simulink model "fir_col_test"  (Simulink 7.2)
settings: Solver=VariableStepDiscrete  StartTime=0.0  StopTime=100  RelTol=1e-3
libraries: xbsIndex_r4 x23, casper_library_downconverter x4
settings Model: Creator=User  LastModifiedBy=root
settings OptimizationCC: InitFltsAndDblsToZero=on
settings DebuggingCC: SaveWithDisabledLinksMsg=none  SaveWithParameterizedLinksMsg=none

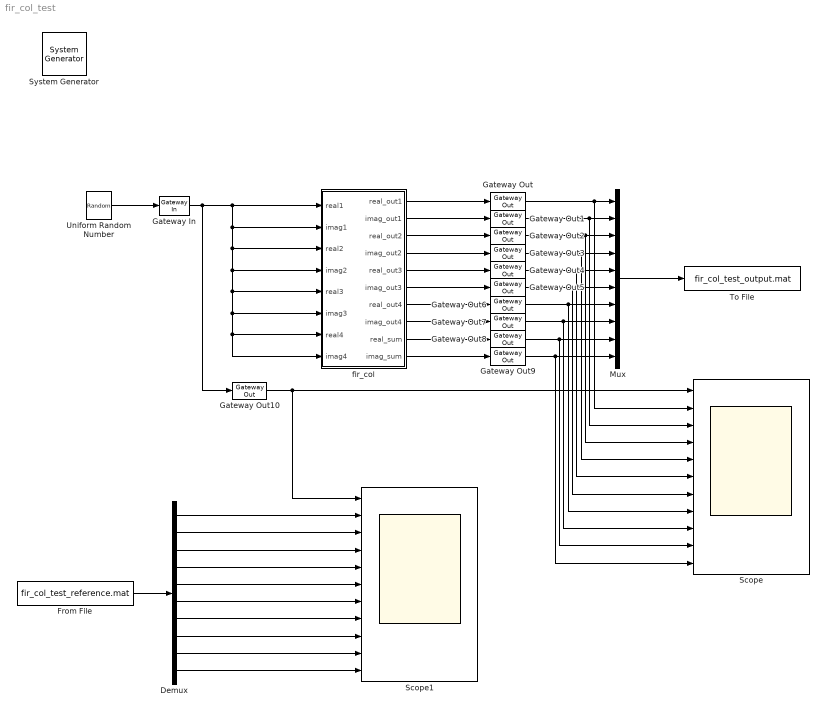
== system fir_col_test ==
  " System Generator" : xbsIndex_r4/ System Generator  Tag=genX  SystemSampleTime=-1  xilinxfamily=Virtex4  part=xc4vsx35  speed=-10  package=ff668  synthesis_tool=XST  clock_wrapper=Clock Enables  directory=./netlist  testbench=off  simulink_period=1  sysclk_period=100  dcm_input_clock_period=100  incr_netlist=off  trim_vbits=Everywhere in SubSystem  dbl_ovrd=According to Block Masks  core_generation=According to Block Masks  run_coregen=off  deprecated_control=off  eval_field=0  block_type=sysgen
      settings: block_version=10.1.1
  Demux : Demux  Outputs=10
  From File : FromFile  FileName=fir_col_test_reference.mat  SampleTime=1
  Gateway In : xbsIndex_r4/Gateway In  arith_type="Signed  (2's comp)"  n_bits=16  bin_pt=15  quantization="Round  (unbiased: +/- Inf)"  overflow=Saturate  period=1  dbl_ovrd=off  timing_constraint=None  locs_specified=off  LOCs={}  hdl_port=on  block_type=gatewayin
      settings: infoedit="Gateway in block.  Converts inputs of type Simulink integer, double and fixed point to  Xilinx fixed point type.<P><P>Hardware notes:  In hardware these blocks become top level input ports."  block_version=10.1.1
  Gateway Out{,1..10} (11 alike) : xbsIndex_r4/Gateway Out  hdl_port=on  timing_constraint=None  locs_specified=off  LOCs={}  block_type=gatewayout
      settings: infoedit="Gateway out block.  Converts Xilinx fixed point inputs into ouputs of type Simulink integer, double, or fixed point.<P><P>Hardware notes:  In hardware these blocks become top level output ports or are discarded, depending on how they are configured."  block_version=10.1.1
  Mux : Mux  Inputs=10
  Scope : Scope  NumInputPorts=11
      settings: YMin=-1~-1~-1~-1~-1~-1~-1~-1~-1~-5~-5  YMax=1~1~1~1~1~1~1~1~1~5~5
  Scope1 : Scope  NumInputPorts=11
      settings: YMin=-1~-1~-1~-1~-1~-1~-1~-1~-1~-5~-5  YMax=1~1~1~1~1~1~1~1~1~5~5
  To File : ToFile  Filename=fir_col_test_output.mat  MatrixName=output
  Uniform Random Number : UniformRandomNumber  SampleTime=0
  fir_col : Subsystem  AncestorBlock=casper_library_downconverter/fir_col  mask(fir_col){n_inputs=4, coeff=getfield( getfield( get_param( gcb,'UserData' ), 'parameters'),'coeff'), add_latency=4, mult_latency=3, coeff_bit_width=18, coeff_bin_pt=17, first_stage_hdl=on, adder_imp=Fabric}
      mask prompts: n_inputs "Inputs"; coeff "Coefficients"; add_latency "Add latency"; mult_latency "Mult Latency"; coeff_bit_width "Coefficient bit width"; coeff_bin_pt "Coefficient binary point"; first_stage_hdl "Implement first stage of adder trees on output as behavioural HDL"; adder_imp "Adder implementation"
      mask init:
      | fir_col_init(gcb, ...
      |     'n_inputs', n_inputs,...
      |     'coeff', coeff, ...
      |     'mult_latency', mult_latency, ...
      |     'add_latency', add_latency, ...
      |     'coeff_bit_width', coeff_bit_width, ...
      |     'coeff_bin_pt', coeff_bin_pt, ...
      |     'first_stage_hdl', first_stage_hdl, ...
      |     'adder_imp', adder_imp);
      mask Help: eval('xlWeb(''http://casper.berkeley.edu/wiki/Fir_col'')')
      mask StyleString: edit,edit,edit,edit,edit,edit,checkbox,popup(Behavioral|Fabric|DSP48)
  wires:
  Uniform Random Number/1 -> Gateway In/1
  Gateway In/1 -> fir_col/8(imag4), fir_col/7(real4), fir_col/6(imag3), fir_col/5(real3), fir_col/4(imag2), fir_col/3(real2), fir_col/2(imag1), fir_col/1(real1), Gateway Out10/1
  fir_col/1(real_out1) -> Gateway Out/1
  fir_col/2(imag_out1) -> Gateway Out1/1
  fir_col/3(real_out2) -> Gateway Out2/1
  fir_col/4(imag_out2) -> Gateway Out3/1
  fir_col/5(real_out3) -> Gateway Out4/1
  fir_col/6(imag_out3) -> Gateway Out5/1
  fir_col/7(real_out4) -> Gateway Out6/1
  fir_col/8(imag_out4) -> Gateway Out7/1
  fir_col/9(real_sum) -> Gateway Out8/1
  fir_col/10(imag_sum) -> Gateway Out9/1
  Gateway Out/1 -> Mux/1, Scope/2
  Gateway Out1/1 -> Mux/2, Scope/3
  Gateway Out2/1 -> Mux/3, Scope/4
  Gateway Out3/1 -> Mux/4, Scope/5
  Gateway Out4/1 -> Mux/5, Scope/6
  Gateway Out5/1 -> Mux/6, Scope/7
  Gateway Out6/1 -> Mux/7, Scope/8
  Gateway Out7/1 -> Mux/8, Scope/9
  Gateway Out8/1 -> Mux/9, Scope/10
  Gateway Out9/1 -> Mux/10, Scope/11
  Mux/1 -> To File/1
  Gateway Out10/1 -> Scope/1, Scope1/1
  From File/1 -> Demux/1
  Demux/1 -> Scope1/2
  Demux/2 -> Scope1/3
  Demux/3 -> Scope1/4
  Demux/4 -> Scope1/5
  Demux/5 -> Scope1/6
  Demux/6 -> Scope1/7
  Demux/7 -> Scope1/8
  Demux/8 -> Scope1/9
  Demux/9 -> Scope1/10
  Demux/10 -> Scope1/11

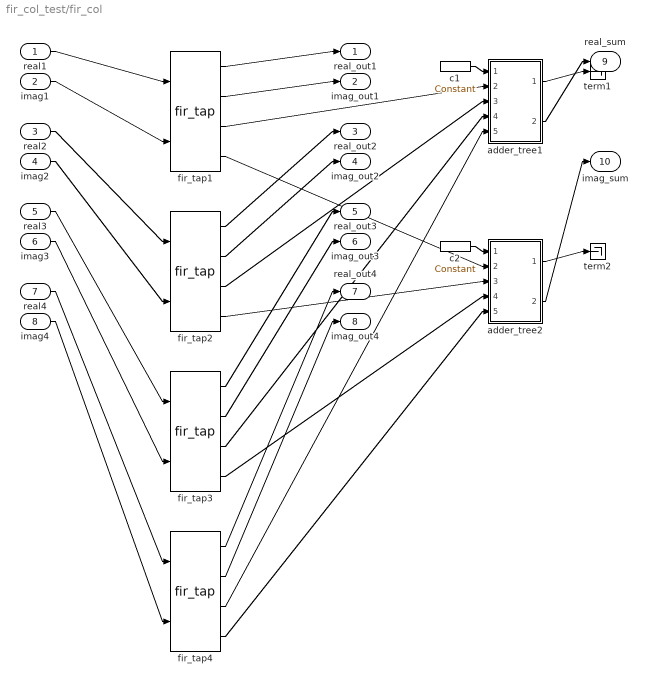
== system fir_col_test/fir_col ==
  real1 : Inport
  imag1 : Inport  Port=2
  real2 : Inport  Port=3
  imag2 : Inport  Port=4
  real3 : Inport  Port=5
  imag3 : Inport  Port=6
  real4 : Inport  Port=7
  imag4 : Inport  Port=8
  adder_tree1 : Subsystem  AncestorBlock=casper_library_misc/adder_tree  mask(adder_tree){n_inputs=4, latency=4, adder_imp=Fabric, first_stage_hdl=on}
      mask prompts: n_inputs "Number of Inputs"; latency "Add Latency"; adder_imp "Adder implementation"; first_stage_hdl "Use behavioural HDL for first stage of adders"
      mask help:
      | Sums all inputs using a tree of adds and delays.
      |
      | Number of inputs: The number of inputs to the block to be summed
      | Add latency: The number of clock cycles to perform one addition (affects timing)..
      | Adder implementation: choice of fabric or DSP48E core, or behavioral HDL
      | Use behavioural HDL for first stage of adders: Causes the first stage of adders to be absorbed into DSP blocks if multipliers precede them (Virtex 5). Overrides Adder implementation
      mask init:
      | adder_tree_init(gcb, ...
      |     'n_inputs', n_inputs, ...
      |     'latency', latency, ...
      |     'adder_imp', adder_imp, ...
      |     'first_stage_hdl', first_stage_hdl);
      settings: AttributesFormatString=latency 8
      mask Help: eval('xlWeb(''http://casper.berkeley.edu/wiki/Adder_tree'')')
      mask StyleString: edit,edit,popup(Behavioral|Fabric|DSP48),checkbox
  adder_tree2 : Subsystem  AncestorBlock=casper_library_misc/adder_tree  mask(adder_tree){n_inputs=4, latency=4, adder_imp=Fabric, first_stage_hdl=on}
      mask prompts: n_inputs "Number of Inputs"; latency "Add Latency"; adder_imp "Adder implementation"; first_stage_hdl "Use behavioural HDL for first stage of adders"
      mask help:
      | Sums all inputs using a tree of adds and delays.
      |
      | Number of inputs: The number of inputs to the block to be summed
      | Add latency: The number of clock cycles to perform one addition (affects timing)..
      | Adder implementation: choice of fabric or DSP48E core, or behavioral HDL
      | Use behavioural HDL for first stage of adders: Causes the first stage of adders to be absorbed into DSP blocks if multipliers precede them (Virtex 5). Overrides Adder implementation
      mask init:
      | adder_tree_init(gcb, ...
      |     'n_inputs', n_inputs, ...
      |     'latency', latency, ...
      |     'adder_imp', adder_imp, ...
      |     'first_stage_hdl', first_stage_hdl);
      settings: AttributesFormatString=latency 8
      mask Help: eval('xlWeb(''http://casper.berkeley.edu/wiki/Adder_tree'')')
      mask StyleString: edit,edit,popup(Behavioral|Fabric|DSP48),checkbox
  c1 : xbsIndex_r4/Constant  arith_type=Signed (2's comp)  const=1  n_bits=16  bin_pt=14  explicit_period=on  period=1  equ=P=C  opselect=C  inp2=PCIN>>17  opr=+  inp1=P  carry=CIN  dbl_ovrd=off  block_type=constant
      settings: block_version=11.4
  c2 : xbsIndex_r4/Constant  arith_type=Signed (2's comp)  const=1  n_bits=16  bin_pt=14  explicit_period=on  period=1  equ=P=C  opselect=C  inp2=PCIN>>17  opr=+  inp1=P  carry=CIN  dbl_ovrd=off  block_type=constant
      settings: block_version=11.4
  fir_tap1 : casper_library_downconverter/fir_tap  SystemSampleTime=-1  factor=0.1  latency=3  coeff_bit_width=18  coeff_bin_pt=17
  fir_tap2 : casper_library_downconverter/fir_tap  SystemSampleTime=-1  factor=0.2  latency=3  coeff_bit_width=18  coeff_bin_pt=17
  fir_tap3 : casper_library_downconverter/fir_tap  SystemSampleTime=-1  factor=0.3  latency=3  coeff_bit_width=18  coeff_bin_pt=17
  fir_tap4 : casper_library_downconverter/fir_tap  SystemSampleTime=-1  factor=0.4  latency=3  coeff_bit_width=18  coeff_bin_pt=17
  term1 : Terminator
  term2 : Terminator
  real_out1 : Outport
  imag_out1 : Outport  Port=2
  real_out2 : Outport  Port=3
  imag_out2 : Outport  Port=4
  real_out3 : Outport  Port=5
  imag_out3 : Outport  Port=6
  real_out4 : Outport  Port=7
  imag_out4 : Outport  Port=8
  real_sum : Outport  Port=9
  imag_sum : Outport  Port=10
  wires:
  adder_tree1/1(sync_out) -> term1/1
  adder_tree2/1(sync_out) -> term2/1
  c1/1 -> adder_tree1/1(sync)
  c2/1 -> adder_tree2/1(sync)
  adder_tree1/2(dout) -> real_sum/1
  adder_tree2/2(dout) -> imag_sum/1
  real1/1 -> fir_tap1/1
  imag1/1 -> fir_tap1/2
  fir_tap1/1 -> real_out1/1
  fir_tap1/2 -> imag_out1/1
  fir_tap1/3 -> adder_tree1/2(din1)
  fir_tap1/4 -> adder_tree2/2(din1)
  real2/1 -> fir_tap2/1
  imag2/1 -> fir_tap2/2
  fir_tap2/1 -> real_out2/1
  fir_tap2/2 -> imag_out2/1
  fir_tap2/3 -> adder_tree1/3(din2)
  fir_tap2/4 -> adder_tree2/3(din2)
  real3/1 -> fir_tap3/1
  imag3/1 -> fir_tap3/2
  fir_tap3/1 -> real_out3/1
  fir_tap3/2 -> imag_out3/1
  fir_tap3/3 -> adder_tree1/4(din3)
  fir_tap3/4 -> adder_tree2/4(din3)
  real4/1 -> fir_tap4/1
  imag4/1 -> fir_tap4/2
  fir_tap4/1 -> real_out4/1
  fir_tap4/2 -> imag_out4/1
  fir_tap4/3 -> adder_tree1/5(din4)
  fir_tap4/4 -> adder_tree2/5(din4)

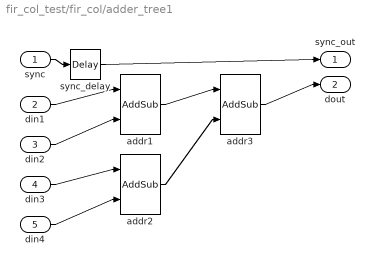
== system fir_col_test/fir_col/adder_tree1 ==
  sync : Inport
  din1 : Inport  Port=2
  din2 : Inport  Port=3
  din3 : Inport  Port=4
  din4 : Inport  Port=5
  addr1 : xbsIndex_r4/AddSub  mode=Addition  use_carryin=off  use_carryout=off  en=off  latency=4  precision=Full  arith_type=Unsigned  n_bits=16  bin_pt=14  quantization=Truncate  overflow=Wrap  dbl_ovrd=off  use_behavioral_HDL=on  hw_selection=Fabric  pipelined=on  use_rpm=on  block_type=addsub
  addr2 : xbsIndex_r4/AddSub  mode=Addition  use_carryin=off  use_carryout=off  en=off  latency=4  precision=Full  arith_type=Unsigned  n_bits=16  bin_pt=14  quantization=Truncate  overflow=Wrap  dbl_ovrd=off  use_behavioral_HDL=on  hw_selection=Fabric  pipelined=on  use_rpm=on  block_type=addsub
  addr3 : xbsIndex_r4/AddSub  mode=Addition  use_carryin=off  use_carryout=off  en=off  latency=4  precision=Full  arith_type=Unsigned  n_bits=16  bin_pt=14  quantization=Truncate  overflow=Wrap  dbl_ovrd=off  use_behavioral_HDL=off  hw_selection=Fabric  pipelined=on  use_rpm=on  block_type=addsub
  sync_delay : xbsIndex_r4/Delay  en=off  latency=8  dbl_ovrd=off  reg_retiming=on  block_type=delay
      settings: block_version=11.4
  sync_out : Outport
  dout : Outport  Port=2
  wires:
  sync/1 -> sync_delay/1
  sync_delay/1 -> sync_out/1
  din1/1 -> addr1/1
  din2/1 -> addr1/2
  din3/1 -> addr2/1
  din4/1 -> addr2/2
  addr1/1 -> addr3/1
  addr2/1 -> addr3/2
  addr3/1 -> dout/1

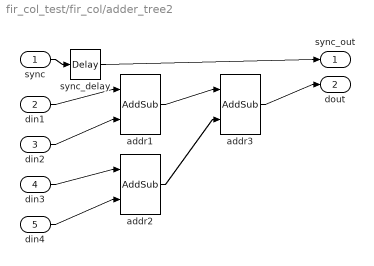
== system fir_col_test/fir_col/adder_tree2 ==
  sync : Inport
  din1 : Inport  Port=2
  din2 : Inport  Port=3
  din3 : Inport  Port=4
  din4 : Inport  Port=5
  addr1 : xbsIndex_r4/AddSub  mode=Addition  use_carryin=off  use_carryout=off  en=off  latency=4  precision=Full  arith_type=Unsigned  n_bits=16  bin_pt=14  quantization=Truncate  overflow=Wrap  dbl_ovrd=off  use_behavioral_HDL=on  hw_selection=Fabric  pipelined=on  use_rpm=on  block_type=addsub
  addr2 : xbsIndex_r4/AddSub  mode=Addition  use_carryin=off  use_carryout=off  en=off  latency=4  precision=Full  arith_type=Unsigned  n_bits=16  bin_pt=14  quantization=Truncate  overflow=Wrap  dbl_ovrd=off  use_behavioral_HDL=on  hw_selection=Fabric  pipelined=on  use_rpm=on  block_type=addsub
  addr3 : xbsIndex_r4/AddSub  mode=Addition  use_carryin=off  use_carryout=off  en=off  latency=4  precision=Full  arith_type=Unsigned  n_bits=16  bin_pt=14  quantization=Truncate  overflow=Wrap  dbl_ovrd=off  use_behavioral_HDL=off  hw_selection=Fabric  pipelined=on  use_rpm=on  block_type=addsub
  sync_delay : xbsIndex_r4/Delay  en=off  latency=8  dbl_ovrd=off  reg_retiming=on  block_type=delay
      settings: block_version=11.4
  sync_out : Outport
  dout : Outport  Port=2
  wires:
  sync/1 -> sync_delay/1
  sync_delay/1 -> sync_out/1
  din1/1 -> addr1/1
  din2/1 -> addr1/2
  din3/1 -> addr2/1
  din4/1 -> addr2/2
  addr1/1 -> addr3/1
  addr2/1 -> addr3/2
  addr3/1 -> dout/1
